simulink model "wattcredit_hw_slow"  (R2023a)
settings: Solver=FixedStepDiscrete  StartTime=0.0  StopTime=hw.sc.stop  FixedStep=Tp  RelTol=1e-3
undefined symbols (not defined in the file or in its folder): hw, Tp
libraries: spsSeriesRLCBranchLib x3, spsDiodeLib x2, spsVoltageMeasurementLib x2, spsCurrentMeasurementLib x1, spsDCVoltageSourceLib x1, spsIdealSwitchLib x1, spspowerguiLib x1
settings Model: Creator=ruthm  LastModifiedBy=ruthm

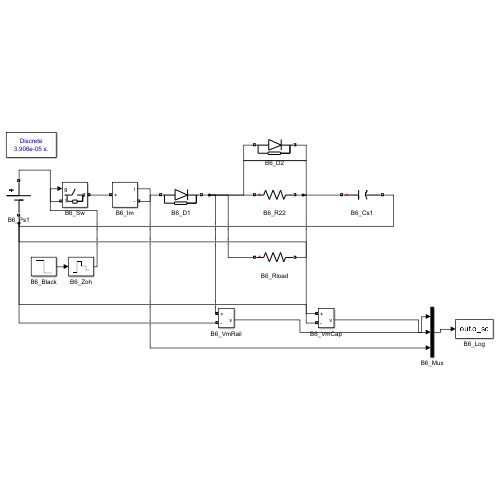
[thumbnail: Simulink's stored preview of the top-level diagram]
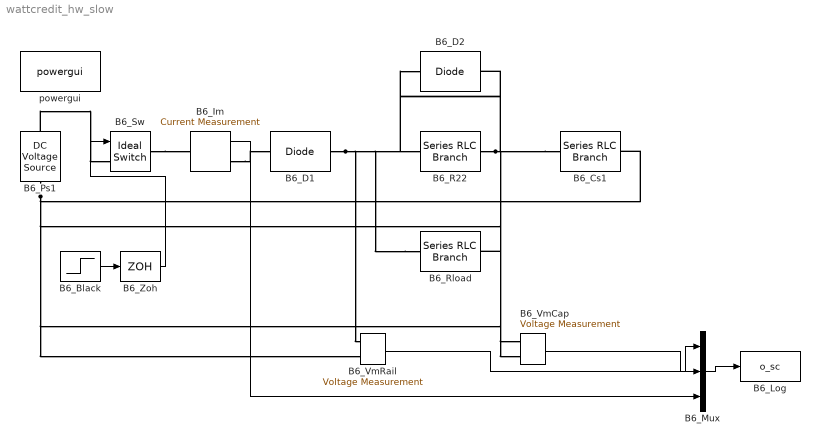
== system wattcredit_hw_slow ==
  B6_Black : Step  Time=hw.sc.tblack  Before=1  After=0  SampleTime=0
  B6_Cs1 : spsSeriesRLCBranchLib/Series RLC Branch  LConnTagsString=__new0  RConnTagsString=__new0  BranchType=C  Resistance=1  Inductance=1e-3  SetiL0=off  InitialCurrent=0  Capacitance=0.1  Setx0=on  InitialVoltage=0  Measurements=None
  B6_D1 : spsDiodeLib/Diode  Ron=hw.sc.Ron  Lon=0  Vf=hw.sc.Vf  IC=0  UseSnubber=0  Rs=500  Cs=250e-9  Measurements=off
  B6_D2 : spsDiodeLib/Diode  Ron=hw.sc.Ron  Lon=0  Vf=hw.sc.Vf  IC=0  UseSnubber=0  Rs=500  Cs=250e-9  Measurements=off
  B6_Im : spsCurrentMeasurementLib/Current Measurement  PhasorSimulation=off  OutputType=Complex  PSBequivalent=0
  B6_Log : ToWorkspace  VariableName=o_sc  SampleTime=-1
      settings: Decimation=100
  B6_Mux : Mux  Inputs=3
  B6_Ps1 : spsDCVoltageSourceLib/DC Voltage Source  Amplitude=hw.sc.Vps  Measurements=None
  B6_R22 : spsSeriesRLCBranchLib/Series RLC Branch  LConnTagsString=__new0  RConnTagsString=__new0  BranchType=R  Resistance=hw.sc.Rchg  Inductance=1e-3  SetiL0=off  InitialCurrent=0  Capacitance=1e-6  Setx0=off  InitialVoltage=0  Measurements=None
  B6_Rload : spsSeriesRLCBranchLib/Series RLC Branch  LConnTagsString=__new0  RConnTagsString=__new0  BranchType=R  Resistance=hw.sc.Rload  Inductance=1e-3  SetiL0=off  InitialCurrent=0  Capacitance=1e-6  Setx0=off  InitialVoltage=0  Measurements=None
  B6_Sw : spsIdealSwitchLib/Ideal Switch  Ron=1e-3  Lon=0  IC=0  Rs=1e6  Cs=inf  Measurements=off
  B6_VmCap : spsVoltageMeasurementLib/Voltage Measurement  PhasorSimulation=off  OutputType=Complex  PSBequivalent=0
  B6_VmRail : spsVoltageMeasurementLib/Voltage Measurement  PhasorSimulation=off  OutputType=Complex  PSBequivalent=0
  B6_Zoh : ZeroOrderHold  SampleTime=3.9063e-05
  powergui : spspowerguiLib/powergui  Priority=1  SimulationMode=Discrete  SampleTime=Tp  frequency=60  Iterations=50  frequencyindice=60  Pbase=100e6  ErrMax=1e-4  UnitsV=kV  UnitsW=MW  buscounter=0  FunctionMessages=off  echomessages=off  EnableUseOfTLC=off  CurrentSourceSwitches=off  DisableSnubberDevices=off  DisableRonSwitches=off  DisableVfSwitches=off  DisplayEquations=off  AutomaticDiscreteSolvers=off  SolverType=Tustin/Backward Euler (TBE)  Interpol=off  ExternalGateDelay=off  methode=off  Ts=100  x0status=blocks  SPID=on  SwTol=0  HookPort=off  NonlinearTolerance=1e-4  nMaxIteration=100  ContinueOnMaxIteration=off  RestoreLinks=warning  ResistiveCurrentMeasurement=off  Frange=[0:2:500]  Ylog=off  Xlog=on  ShowGrid=off  save=off  variable=ZData  structure=0  ZoomFFT=off  StartTime=0.0  cycles=1  DisplayStyle=1  fundamental=60  FreqAxis=off  MaxFrequency=1000  frequencyindicesteady=1  RmsSteady=1  display=off
  wires:
  B6_Black/1 -> B6_Zoh/1
  B6_Zoh/1 -> B6_Sw/1
  B6_VmRail/1 -> B6_Mux/1
  B6_VmCap/1 -> B6_Mux/2
  B6_Im/1 -> B6_Mux/3
  B6_Mux/1 -> B6_Log/1
  connections:
  B6_Ps1/RConn1 -- B6_Sw/LConn1
  B6_Sw/RConn1 -- B6_Im/LConn1
  B6_Im/RConn1 -- B6_D1/LConn1
  B6_Rload/LConn1 -- B6_D1/RConn1 -- B6_R22/LConn1 -- B6_D2/RConn1 -- B6_VmRail/LConn1
  B6_Cs1/LConn1 -- B6_R22/RConn1 -- B6_D2/LConn1 -- B6_VmCap/LConn1
  B6_Rload/RConn1 -- B6_Ps1/LConn1 -- B6_Cs1/RConn1 -- B6_VmRail/LConn2 -- B6_VmCap/LConn2
